simulink model "hopper_6dof_NED_v2_fswBridge"  (R2026a)
settings: Solver=FixedStepAuto  StopTime=30  FixedStep=1e-3  RelTol=1e-5
InitFcn:
  | if ~exist('SENS', 'var'), addpath(fullfile(fileparts(get_param(bdroot, 'FileName')), 'fsw_bridge')); SENS = sensor_params(); end
undefined symbols (not defined in the file): cg_init, dcg_dMfu_table, dcg_dMox_table, dI_dMfu_table, dI_dMox_table, ENGINE, engine_cg, engine_mass, fu_axial_damping_ratios, fu_lateral_damping_ratios, fu_mass_profile, fu_masses, fu_mdot_data, g, IN, K1flat, K2grid, MoI_init, mount_cg, OUT, ox_axial_damping_ratios, ox_lateral_damping_ratios, ox_mass_profile, ox_masses, ox_mdot_data, pressureLevels, r_leg_1, r_leg_2, r_leg_3, r_leg_4, tank_r, TANKS, Target_Trajectory, tgrid, thrust_data, unom, uwndTable, VEH, vwndTable
libraries: fl_lib x31, nesl_utility x25, matrix_library x18, SimscapeFluids_lib x10, simulink_extras x7, slpidlib x7, simulink x5, dspindex x3, sl_discontinuities x2, aerolibanim x1, commrandsrc3 x1, aerolibutil x1
(part 7 of 7)

== system hopper_6dof_NED_v2_fswBridge/Environment/Ground /Leg 1 Force2/If Action Subsystem ==
  Leg Position : Inport
  Leg Velocity : Inport  Port=2
  Action Port : ActionPort  ActionPortLabel=|
      | if(u1 > -0.001 
      | )
  Constant : Constant  Value=0.001
  Demux : Demux  Outputs=3
  Demux1 : Demux  Outputs=3
  Divide : Product  Inputs=*/
  Dot Product : DotProduct  OutDataTypeStr=Inherit: Inherit via internal rule
  Gain : Gain  Gain=-147150
  Gain1 : Gain  Gain=-7672.03
  Gain2 : Gain  Gain=-0.6
  Gain3 : Gain  Gain=-1
  Gain4 : Gain  Gain=-1
  Mux : Mux  Inputs=3
  Mux1 : Mux  Inputs=3
  Product : Product
  Sqrt : Sqrt
  Sum : Sum  Inputs=|++
  Sum1 : Sum  Inputs=|++
  Sum2 : Sum  Inputs=|++
  Zero : Constant  Value=0  OutDataTypeStr=Inherit: Inherit via back propagation
  Zero1 : Constant  Value=0  OutDataTypeStr=Inherit: Inherit via back propagation
  Zero2 : Constant  Value=0  OutDataTypeStr=Inherit: Inherit via back propagation
  Leg Force : Outport
  wires:
  Leg Position/1 -> Demux/1
  Leg Velocity/1 -> Demux1/1
  Gain/1 -> Sum/1
  Gain1/1 -> Sum/2
  Demux1/3 -> Gain1/1
  Demux1/2 -> Mux/2
  Demux1/1 -> Mux/1
  Mux/1 -> Dot Product/2, Dot Product/1, Divide/1
  Dot Product/1 -> Sqrt/1
  Divide/1 -> Product/2
  Gain2/1 -> Product/1
  Product/1 -> Gain4/1
  Sum1/1 -> Leg Force/1
  Sqrt/1 -> Sum2/1
  Sum2/1 -> Divide/2
  Constant/1 -> Sum2/2
  Sum/1 -> Gain3/1
  Zero1/1 -> Mux1/2
  Zero2/1 -> Mux1/3
  Mux1/1 -> Sum1/1, Gain2/1
  Demux/3 -> Gain/1
  Zero/1 -> Mux/3
  Gain3/1 -> Mux1/1
  Gain4/1 -> Sum1/2

== system hopper_6dof_NED_v2_fswBridge/Environment/Ground /Leg 1 Force2/If Action Subsystem1 ==
  Action Port : ActionPort  ActionPortLabel=else
  Constant : Constant  Value=[0 0 0]
  Out1 : Outport
  wires:
  Constant/1 -> Out1/1

== system hopper_6dof_NED_v2_fswBridge/Environment/Ground /Leg 1 Force3/If Action Subsystem ==
  Leg Position : Inport
  Leg Velocity : Inport  Port=2
  Action Port : ActionPort  ActionPortLabel=|
      | if(u1 > -0.001 
      | )
  Constant : Constant  Value=0.001
  Demux : Demux  Outputs=3
  Demux1 : Demux  Outputs=3
  Divide : Product  Inputs=*/
  Dot Product : DotProduct  OutDataTypeStr=Inherit: Inherit via internal rule
  Gain : Gain  Gain=-147150
  Gain1 : Gain  Gain=-7672.03
  Gain2 : Gain  Gain=-0.6
  Gain3 : Gain  Gain=-1
  Gain4 : Gain  Gain=-1
  Mux : Mux  Inputs=3
  Mux1 : Mux  Inputs=3
  Product : Product
  Sqrt : Sqrt
  Sum : Sum  Inputs=|++
  Sum1 : Sum  Inputs=|++
  Sum2 : Sum  Inputs=|++
  Zero : Constant  Value=0  OutDataTypeStr=Inherit: Inherit via back propagation
  Zero1 : Constant  Value=0  OutDataTypeStr=Inherit: Inherit via back propagation
  Zero2 : Constant  Value=0  OutDataTypeStr=Inherit: Inherit via back propagation
  Leg Force : Outport
  wires:
  Leg Position/1 -> Demux/1
  Leg Velocity/1 -> Demux1/1
  Gain/1 -> Sum/1
  Gain1/1 -> Sum/2
  Demux1/3 -> Gain1/1
  Demux1/2 -> Mux/2
  Demux1/1 -> Mux/1
  Mux/1 -> Dot Product/2, Dot Product/1, Divide/1
  Dot Product/1 -> Sqrt/1
  Divide/1 -> Product/2
  Gain2/1 -> Product/1
  Product/1 -> Gain4/1
  Sum1/1 -> Leg Force/1
  Sqrt/1 -> Sum2/1
  Sum2/1 -> Divide/2
  Constant/1 -> Sum2/2
  Sum/1 -> Gain3/1
  Zero1/1 -> Mux1/2
  Zero2/1 -> Mux1/3
  Mux1/1 -> Sum1/1, Gain2/1
  Demux/3 -> Gain/1
  Zero/1 -> Mux/3
  Gain3/1 -> Mux1/1
  Gain4/1 -> Sum1/2

== system hopper_6dof_NED_v2_fswBridge/Environment/Ground /Leg 1 Force3/If Action Subsystem1 ==
  Action Port : ActionPort  ActionPortLabel=else
  Constant : Constant  Value=[0 0 0]
  Out1 : Outport
  wires:
  Constant/1 -> Out1/1

== matlab function hopper_6dof_NED_v2_fswBridge/Environment/Slosh/Oxidizer Yaw Force/MATLAB Function ==
  data: ox_yaw_accel input; accel_term output; ox_lateral_pendulum_l input
function accel_term = fcn(ox_yaw_accel, ox_lateral_pendulum_l)

accel_term = -ox_yaw_accel / ox_lateral_pendulum_l;

end

== matlab function hopper_6dof_NED_v2_fswBridge/Environment/Slosh/Oxidizer Yaw Force/MATLAB Function1 ==
  data: ox_yaw_phi input; ang_term output; ox_lateral_natural_freq input
function ang_term = fcn(ox_yaw_phi, ox_lateral_natural_freq)

ang_term = -ox_lateral_natural_freq^2 * ox_yaw_phi;

end

== matlab function hopper_6dof_NED_v2_fswBridge/Environment/Slosh/Oxidizer Yaw Force/MATLAB Function2 ==
  data: ox_yaw_phi_dot input; velo_term output; ox_lateral_natural_freq input; ox_lateral_damping input
function velo_term = fcn(ox_yaw_phi_dot, ox_lateral_natural_freq,ox_lateral_damping)

velo_term = -2 * ox_lateral_damping * ox_lateral_natural_freq * ox_yaw_phi_dot;
end

== matlab function hopper_6dof_NED_v2_fswBridge/Environment/Slosh/Oxidizer Yaw Force/MATLAB Function3 ==
  data: ox_yaw_phi_ddot input; ox_yaw_f output; ox_lateral_slosh_mass input; ox_lateral_pendulum_l input
function ox_yaw_f = fcn(ox_yaw_phi_ddot, ox_lateral_slosh_mass, ox_lateral_pendulum_l)

ox_yaw_f = ox_lateral_slosh_mass * ox_lateral_pendulum_l * ox_yaw_phi_ddot;
end

== matlab function hopper_6dof_NED_v2_fswBridge/Environment/Slosh/Oxidizer Axial Force/MATLAB Function ==
  data: ox_axial_accel input; accel_term output; ox_axial_pendulum_l input
function accel_term = fcn(ox_axial_accel, ox_axial_pendulum_l)

accel_term = -ox_axial_accel / ox_axial_pendulum_l;

end

== matlab function hopper_6dof_NED_v2_fswBridge/Environment/Slosh/Oxidizer Axial Force/MATLAB Function1 ==
  data: ox_axial_phi input; ang_term output; ox_axial_natural_freq input
function ang_term = fcn(ox_axial_phi, ox_axial_natural_freq)

ang_term = -ox_axial_natural_freq^2 * ox_axial_phi;

end

== matlab function hopper_6dof_NED_v2_fswBridge/Environment/Slosh/Oxidizer Axial Force/MATLAB Function2 ==
  data: ox_axial_phi_dot input; velo_term output; ox_axial_natural_freq input; ox_axial_damping input
function velo_term = fcn(ox_axial_phi_dot, ox_axial_natural_freq,ox_axial_damping)

velo_term = -2 * ox_axial_damping * ox_axial_natural_freq * ox_axial_phi_dot;
end

== matlab function hopper_6dof_NED_v2_fswBridge/Environment/Slosh/Oxidizer Axial Force/MATLAB Function3 ==
  data: ox_axial_phi_ddot input; ox_axial_f output; ox_axial_slosh_mass input; ox_axial_pendulum_l input
function ox_axial_f = fcn(ox_axial_phi_ddot, ox_axial_slosh_mass, ox_axial_pendulum_l)

ox_axial_f = ox_axial_slosh_mass * ox_axial_pendulum_l * ox_axial_phi_ddot;
end

== matlab function hopper_6dof_NED_v2_fswBridge/Environment/Slosh/Fuel Axial Force/MATLAB Function ==
  data: fu_axial_accel input; accel_term output; fu_axial_pendulum_l input
function accel_term = fcn(fu_axial_accel, fu_axial_pendulum_l)

accel_term = -fu_axial_accel / fu_axial_pendulum_l;

end

== matlab function hopper_6dof_NED_v2_fswBridge/Environment/Slosh/Fuel Axial Force/MATLAB Function1 ==
  data: fu_axial_phi input; ang_term output; fu_axial_natural_freq input
function ang_term = fcn(fu_axial_phi, fu_axial_natural_freq)

ang_term = -fu_axial_natural_freq^2 * fu_axial_phi;

end

== matlab function hopper_6dof_NED_v2_fswBridge/Environment/Slosh/Fuel Axial Force/MATLAB Function2 ==
  data: fu_axial_phi_dot input; velo_term output; fu_axial_natural_freq input; fu_axial_damping input
function velo_term = fcn(fu_axial_phi_dot, fu_axial_natural_freq,fu_axial_damping)

velo_term = -2 * fu_axial_damping * fu_axial_natural_freq * fu_axial_phi_dot;
end

== matlab function hopper_6dof_NED_v2_fswBridge/Environment/Slosh/Fuel Axial Force/MATLAB Function3 ==
  data: fu_axial_phi_ddot input; fu_axial_f output; fu_axial_slosh_mass input; fu_axial_pendulum_l input
function fu_axial_f = fcn(fu_axial_phi_ddot, fu_axial_slosh_mass, fu_axial_pendulum_l)

fu_axial_f = fu_axial_slosh_mass * fu_axial_pendulum_l * fu_axial_phi_ddot;
end

== matlab function hopper_6dof_NED_v2_fswBridge/Environment/Slosh/Fuel Yaw Force/MATLAB Function ==
  data: fu_pitch_accel input; accel_term output; fu_lateral_pendulum_l input
function accel_term = fcn(fu_pitch_accel, fu_lateral_pendulum_l)

accel_term = -fu_pitch_accel / fu_lateral_pendulum_l;

end

== matlab function hopper_6dof_NED_v2_fswBridge/Environment/Slosh/Fuel Yaw Force/MATLAB Function1 ==
  data: fu_pitch_phi input; ang_term output; fu_lateral_natural_freq input
function ang_term = fcn(fu_pitch_phi, fu_lateral_natural_freq)

ang_term = -fu_lateral_natural_freq^2 * fu_pitch_phi;

end

== matlab function hopper_6dof_NED_v2_fswBridge/Environment/Slosh/Fuel Yaw Force/MATLAB Function2 ==
  data: fu_pitch_phi_dot input; velo_term output; fu_lateral_natural_freq input; fu_lateral_damping input
function velo_term = fcn(fu_pitch_phi_dot, fu_lateral_natural_freq,fu_lateral_damping)

velo_term = -2 * fu_lateral_damping * fu_lateral_natural_freq * fu_pitch_phi_dot;
end

== matlab function hopper_6dof_NED_v2_fswBridge/Environment/Slosh/Fuel Yaw Force/MATLAB Function3 ==
  data: fu_pitch_phi_ddot input; fu_pitch_f output; fu_lateral_slosh_mass input; fu_lateral_pendulum_l input
function fu_pitch_f = fcn(fu_pitch_phi_ddot, fu_lateral_slosh_mass, fu_lateral_pendulum_l)

fu_pitch_f = fu_lateral_slosh_mass * fu_lateral_pendulum_l * fu_pitch_phi_ddot;
end

== matlab function hopper_6dof_NED_v2_fswBridge/Environment/Slosh/Fuel Pitch Force/MATLAB Function ==
  data: fu_yaw_accel input; accel_term output; fu_lateral_pendulum_l input
function accel_term = fcn(fu_yaw_accel, fu_lateral_pendulum_l)

accel_term = -fu_yaw_accel / fu_lateral_pendulum_l;

end

== matlab function hopper_6dof_NED_v2_fswBridge/Environment/Slosh/MATLAB Function ==
  data: ox_lateral_natural_freq output; ox_axial_natural_freq output; ox_mass input; ox_lateral_slosh_mass output; ox_axial_slosh_mass output; ox_lateral_pendulum_l output; ox_aeff input; ox_axial_pendulum_l output; ox_lateral_damping output; ox_axial_damping output; tank_r input; ox_lateral_damping input; ox_axial_damping input
function [ox_lateral_natural_freq, ox_axial_natural_freq, ox_lateral_slosh_mass,ox_axial_slosh_mass, ox_lateral_pendulum_l, ox_axial_pendulum_l, ox_lateral_damping, ox_axial_damping]  = slosh_parameters(ox_mass, ox_aeff, tank_r, ox_lateral_damping, ox_axial_damping)

zeta = 1.841; % 1st eigen mode of oscillation for a cylindrical tank
ox_density = 1141;   % kg/m^3
% ox_tank_cg = 1.854; % m
% ox_tank_h =  TANKS.singular.oxidizer.h;
geff = norm(ox_aeff) + 0.001;

% Oxidizer Fluid
if ox_mass > 0.001
   h_ox_fluid = (ox_mass / ox_density) / (pi * tank_r^2);

   % Slosh Natural Frequencies
    ox_lateral_natural_freq = sqrt(zeta * geff / tank_r) * tanh(zeta * h_ox_fluid / tank_r);
    ox_axial_natural_freq = pi * sqrt(geff / h_ox_fluid);

    % Slosh Masses 
    ox_lateral_slosh_mass = ox_mass * (2 * tank_r * tanh(2 * zeta * h_ox_fluid / (2 * tank_r))) / (zeta * (zeta^2 - 1) * h_ox_fluid);
    ox_axial_slosh_mass = 1 / (pi^2) *  ox_mass;

    % Slosh Pendulum Lengths
    ox_lateral_pendulum_l = (2 * tank_r) / (2 * zeta * tanh(2*zeta * h_ox_fluid / (2 * tank_r)));
    ox_axial_pendulum_l = geff / ox_axial_natural_freq^2;
else
   h_ox_fluid = 0; 
   ox_lateral_natural_freq = 0;
   ox_axial_natural_freq = 0;
   ox_lateral_slosh_mass = 0;
   ox_axial_slosh_mass = 0;
   ox_lateral_pendulum_l = 1;
   ox_axial_pendulum_l = 1;
end



end

== matlab function hopper_6dof_NED_v2_fswBridge/Environment/Slosh/Fuel Pitch Force/MATLAB Function1 ==
  data: fu_yaw_phi input; ang_term output; fu_lateral_natural_freq input
function ang_term = fcn(fu_yaw_phi, fu_lateral_natural_freq)

ang_term = -fu_lateral_natural_freq^2 * fu_yaw_phi;

end

== matlab function hopper_6dof_NED_v2_fswBridge/Environment/Slosh/Fuel Pitch Force/MATLAB Function2 ==
  data: fu_yaw_phi_dot input; velo_term output; fu_lateral_natural_freq input; fu_lateral_damping input
function velo_term = fcn(fu_yaw_phi_dot, fu_lateral_natural_freq, fu_lateral_damping)

velo_term = -2 * fu_lateral_damping * fu_lateral_natural_freq * fu_yaw_phi_dot;
end

== matlab function hopper_6dof_NED_v2_fswBridge/Environment/Slosh/Fuel Pitch Force/MATLAB Function3 ==
  data: fu_yaw_phi_ddot input; fu_yaw_f output; fu_lateral_slosh_mass input; fu_lateral_pendulum_l input
function fu_yaw_f = fcn(fu_yaw_phi_ddot, fu_lateral_slosh_mass, fu_lateral_pendulum_l)

fu_yaw_f = fu_lateral_slosh_mass * fu_lateral_pendulum_l * fu_yaw_phi_ddot;
end

== matlab function hopper_6dof_NED_v2_fswBridge/Environment/CG // MOI Script v3/MATLAB Function ==
  data: r_ox input; I_m_ox output
function I_m_ox = fcn(r_ox)
x = r_ox(1);
y = r_ox(2);
z = r_ox(3);

I_m_ox = [y^2 + z^2 -x*y x*z;
       -x*y x^2 + z^2 -y*z;
       -x*z y*z  x^2 + y^2
    ];

== matlab function hopper_6dof_NED_v2_fswBridge/Environment/CG // MOI Script v3/MATLAB Function1 ==
  data: r_fu input; I_m_fu output
function I_m_fu = fcn(r_fu)
x = r_fu(1);
y = r_fu(2);
z = r_fu(3);

I_m_fu = [y^2 + z^2 -x*y x*z;
       -x*y x^2 + z^2 -y*z;
       -x*z y*z  x^2 + y^2
    ];

== matlab function hopper_6dof_NED_v2_fswBridge/Environment/Slosh/Oxidizer Axial Force/MATLAB Function4 ==
  data: x_omega_dot input; x_slosh_torque output; ox_axial_slosh_mass input; ox_axial_pendulum_l input; slosh_angular_accel input
function x_slosh_torque = fcn(x_omega_dot, ox_axial_slosh_mass, ox_axial_pendulum_l, slosh_angular_accel)

I_s = ox_axial_slosh_mass * ox_axial_pendulum_l^2;

x_slosh_torque = -I_s*(x_omega_dot - slosh_angular_accel);

== matlab function hopper_6dof_NED_v2_fswBridge/Environment/Slosh/Fuel Axial Force/MATLAB Function4 ==
  data: x_omega_dot input; x_slosh_torque output; fu_axial_slosh_mass input; fu_axial_pendulum_l input; slosh_angular_accel input
function x_slosh_torque = fcn(x_omega_dot, fu_axial_slosh_mass, fu_axial_pendulum_l, slosh_angular_accel)

I_s = fu_axial_slosh_mass * fu_axial_pendulum_l^2;

x_slosh_torque = -I_s*(x_omega_dot - slosh_angular_accel);

== matlab function hopper_6dof_NED_v2_fswBridge/Environment/Slosh/Oxidizer Yaw Force/MATLAB Function4 ==
  data: y_omega_dot input; y_slosh_torque output; ox_lateral_slosh_mass input; ox_lateral_pendulum_l input; slosh_angular_accel input
function y_slosh_torque = fcn(y_omega_dot, ox_lateral_slosh_mass, ox_lateral_pendulum_l, slosh_angular_accel)

I_s = ox_lateral_slosh_mass * ox_lateral_pendulum_l^2;

y_slosh_torque = -I_s*(y_omega_dot - slosh_angular_accel);

== matlab function hopper_6dof_NED_v2_fswBridge/Environment/Slosh/Fuel Yaw Force/MATLAB Function4 ==
  data: y_omega_dot input; y_slosh_torque output; fu_lateral_slosh_mass input; fu_lateral_pendulum_l input; slosh_angular_accel input
function y_slosh_torque = fcn(y_omega_dot, fu_lateral_slosh_mass, fu_lateral_pendulum_l, slosh_angular_accel)

I_s = fu_lateral_slosh_mass * fu_lateral_pendulum_l^2;

y_slosh_torque = -I_s*(y_omega_dot - slosh_angular_accel);

== matlab function hopper_6dof_NED_v2_fswBridge/Environment/Slosh/Oxidizer Pitch Force/MATLAB Function4 ==
  data: z_omega_dot input; z_slosh_torque output; ox_lateral_slosh_mass input; ox_lateral_pendulum_l input; slosh_angular_accel input
function z_slosh_torque = fcn(z_omega_dot, ox_lateral_slosh_mass, ox_lateral_pendulum_l, slosh_angular_accel)

I_s = ox_lateral_slosh_mass * ox_lateral_pendulum_l^2;

z_slosh_torque = -I_s*(z_omega_dot - slosh_angular_accel);

== matlab function hopper_6dof_NED_v2_fswBridge/Environment/Slosh/Fuel Pitch Force/MATLAB Function4 ==
  data: z_omega_dot input; z_slosh_torque output; fu_lateral_slosh_mass input; fu_lateral_pendulum_l input; slosh_angular_accel input
function z_slosh_torque = fcn(z_omega_dot, fu_lateral_slosh_mass, fu_lateral_pendulum_l, slosh_angular_accel)

I_s = fu_lateral_slosh_mass * fu_lateral_pendulum_l^2;

z_slosh_torque = -I_s*(z_omega_dot - slosh_angular_accel);

== matlab function hopper_6dof_NED_v2_fswBridge/Environment/CG // MOI Script v3/MATLAB Function2 ==
  data: delta_y input; rot_mat output; delta_z input
function rot_mat = fcn(delta_y, delta_z)

rot_mat = [0 -delta_z delta_y;
           delta_z 0 0;
           -delta_y 0 0];

== matlab function hopper_6dof_NED_v2_fswBridge/Environment/Sensors/imu_model ==
  settings: updateMethod=DISCRETE  sampleTime=SENS.imu.Ts
  data: F_b input; imu output; W_b input; mass input; w_b input; SENS parameter
function imu = imu_model(F_b, W_b, mass, w_b, SENS)
%#codegen
% IMU measurement model (Notion: IMU Measurement Model), ADIS16500.
%   F_b  total force on the vehicle, body axes (N)
%   W_b  weight, body axes (N)
%   mass vehicle mass (kg)
%   w_b  body angular rate (rad/s)
%   imu  [accel (3) m/s^2; gyro (3) deg/s], sensor axes
%
%   f = (I+Ma)(I+Sa) Rbs f_true + ba + na
%   w = (I+Mg)(I+Sg) Rbs w_true + Gg Rbs f_true + bg + ng
%   Biases = turn-on offset (drawn once) + first-order Gauss-Markov drift.
P = SENS.imu;
persistent s ba0 bg0 bad bgd Sa Sg Ma Mg
if isempty(s)
    s = rng_seed(SENS.seed, 1);
    [n, s] = rng_gauss(s, 3); ba0 = P.acc_b0_sd * n;
    [n, s] = rng_gauss(s, 3); bg0 = P.gyro_b0_sd * n;
    [n, s] = rng_gauss(s, 3); bad = P.acc_b_sd * n;
    [n, s] = rng_gauss(s, 3); bgd = P.gyro_b_sd * n;
    [n, s] = rng_gauss(s, 3); Sa = diag(1 + P.sf_sd * n);
    [n, s] = rng_gauss(s, 3); Sg = diag(1 + P.sf_sd * n);
    [n, s] = rng_gauss(s, 6); Ma = eye(3) + P.misalign_sd * [0 n(1) n(2); n(3) 0 n(4); n(5) n(6) 0];
    [n, s] = rng_gauss(s, 6); Mg = eye(3) + P.misalign_sd * [0 n(1) n(2); n(3) 0 n(4); n(5) n(6) 0];
end

% Specific force at the CG, plus centripetal term at the sensor location
f_true = (F_b(:) - W_b(:)) / mass + cross(w_b(:), cross(w_b(:), P.r_b));
f_s = P.R_bs * f_true;
w_s = P.R_bs * w_b(:);

% Gauss-Markov bias drift
phi_a = exp(-P.Ts / P.acc_b_tau);
phi_g = exp(-P.Ts / P.gyro_b_tau);
[n, s] = rng_gauss(s, 3); bad = phi_a * bad + sqrt(1 - phi_a^2) * P.acc_b_sd * n;
[n, s] = rng_gauss(s, 3); bgd = phi_g * bgd + sqrt(1 - phi_g^2) * P.gyro_b_sd * n;

% White noise, per-sample sd from the noise density
[na, s] = rng_gauss(s, 3);
[ng, s] = rng_gauss(s, 3);
f_meas = Ma * Sa * f_s + ba0 + bad + P.acc_nd / sqrt(P.Ts) * na;
w_meas = Mg * Sg * w_s + P.g_sens * f_s + bg0 + bgd + P.gyro_nd / sqrt(P.Ts) * ng;

imu = [f_meas; w_meas * (180 / pi)];
end

% --- deterministic RNG shared by the sensor blocks (xorshift32 + Box-Muller)
% Same numbers in Simulink and in generated C, seeded per run and per sensor.
function s = rng_seed(seed, stream)
s = uint32(mod(double(seed) * 2654435761 + double(stream) * 97531 + 12345, 4294967296));
if s == 0
    s = uint32(1);
end
end

function [u, s] = rng_uniform(s)
s = bitxor(s, bitshift(s, 13));
s = bitxor(s, bitshift(s, -17));
s = bitxor(s, bitshift(s, 5));
u = (double(s) + 0.5) / 4294967296;
end

function [n, s] = rng_gauss(s, k)
n = zeros(k, 1);
for i = 1:k
    [u1, s] = rng_uniform(s);
    [u2, s] = rng_uniform(s);
    n(i) = sqrt(-2 * log(u1)) * cos(2 * pi * u2);
end
end

== matlab function hopper_6dof_NED_v2_fswBridge/Environment/Sensors/mag_model ==
  settings: updateMethod=DISCRETE  sampleTime=SENS.mag.Ts
  data: C_bn input; mag output; SENS parameter
function mag = mag_model(C_bn, SENS)
%#codegen
% Magnetometer measurement model (Notion: Magnetometer Model), LIS2MDL.
%   C_bn NED -> body rotation (6DOF DCMbe)
%   mag  magnetic field, sensor axes, Gauss
%
%   z = A Cbn Bn + beta + eta
%   A folds soft iron, scale factor and misalignment; beta is hard iron.
%   Both are drawn once per run (they are what calibration estimates).
P = SENS.mag;
persistent s A beta
if isempty(s)
    s = rng_seed(SENS.seed, 2);
    [n, s] = rng_gauss(s, 9); A = eye(3) + P.A_sd * reshape(n, 3, 3);
    [n, s] = rng_gauss(s, 3); beta = P.beta_sd * n;
end

[n, s] = rng_gauss(s, 3);
mag = A * (C_bn * P.B_n) + beta + P.noise_sd * n;
end

% --- deterministic RNG shared by the sensor blocks (xorshift32 + Box-Muller)
function s = rng_seed(seed, stream)
s = uint32(mod(double(seed) * 2654435761 + double(stream) * 97531 + 12345, 4294967296));
if s == 0
    s = uint32(1);
end
end

function [u, s] = rng_uniform(s)
s = bitxor(s, bitshift(s, 13));
s = bitxor(s, bitshift(s, -17));
s = bitxor(s, bitshift(s, 5));
u = (double(s) + 0.5) / 4294967296;
end

function [n, s] = rng_gauss(s, k)
n = zeros(k, 1);
for i = 1:k
    [u1, s] = rng_uniform(s);
    [u2, s] = rng_uniform(s);
    n(i) = sqrt(-2 * log(u1)) * cos(2 * pi * u2);
end
end

== matlab function hopper_6dof_NED_v2_fswBridge/Environment/Sensors/baro_model ==
  settings: updateMethod=DISCRETE  sampleTime=SENS.baro.Ts
  data: p_n input; baro output; v_n input; C_bn input; thrust input; SENS parameter
function baro = baro_model(p_n, v_n, C_bn, thrust, SENS)
%#codegen
% Barometer measurement model (Notion: Barometer Model), MS5611.
%   p_n    CG position NED (m), ground at D = 0
%   v_n    CG velocity NED (m/s)
%   C_bn   NED -> body rotation
%   thrust delivered thrust (N); > 0 means the engine is on
%   baro   [pressure Pa; temperature degC]
%
%   p = p_atm(h) + dp_ground_effect(h) + dp_dynamic + beta + eta, quantized
%   Tare/zeroing is left to the flight software.
P = SENS.baro;
persistent s b
if isempty(s)
    s = rng_seed(SENS.seed, 3);
    [n, s] = rng_gauss(s, 1); b = P.b0_sd * n;
end

% Height of the sensor port above the pad
r_n = C_bn' * P.r_b;
h = -(p_n(3) + r_n(3));

% Standard atmosphere from the pad conditions
T = P.T_pad - P.L * h;
p_atm = P.p_pad * (T / P.T_pad)^(P.g0 / (P.L * P.R));

% Exhaust ground effect, only near the pad with the engine on
dp_ge = 0;
if thrust > 0 && h < P.ge_D
    dp_ge = P.ge_sign * P.ge_A * (P.ge_D - max(h, 0))^2;
end

% Part of the dynamic pressure reaching the port
rho = p_atm / (P.R * T);
v_rel = v_n(:) - P.wind_n;
dp_dyn = P.k_port * 0.5 * rho * (v_rel' * v_rel);

% Gauss-Markov bias drift and white noise
phi = exp(-P.Ts / P.b_tau);
[n, s] = rng_gauss(s, 2);
b = phi * b + sqrt(1 - phi^2) * P.b_sd * n(1);
p = p_atm + dp_ge + dp_dyn + b + P.noise_sd * n(2);

baro = [P.dq * round(p / P.dq); T - 273.15];
end

% --- deterministic RNG shared by the sensor blocks (xorshift32 + Box-Muller)
function s = rng_seed(seed, stream)
s = uint32(mod(double(seed) * 2654435761 + double(stream) * 97531 + 12345, 4294967296));
if s == 0
    s = uint32(1);
end
end

function [u, s] = rng_uniform(s)
s = bitxor(s, bitshift(s, 13));
s = bitxor(s, bitshift(s, -17));
s = bitxor(s, bitshift(s, 5));
u = (double(s) + 0.5) / 4294967296;
end

function [n, s] = rng_gauss(s, k)
n = zeros(k, 1);
for i = 1:k
    [u1, s] = rng_uniform(s);
    [u2, s] = rng_uniform(s);
    n(i) = sqrt(-2 * log(u1)) * cos(2 * pi * u2);
end
end

== matlab function hopper_6dof_NED_v2_fswBridge/Environment/Sensors/gps_model ==
  settings: updateMethod=DISCRETE  sampleTime=SENS.gps.tick
  data: p_n input; gps output; v_n input; C_bn input; w_b input; thrust input; SENS parameter
function gps = gps_model(p_n, v_n, C_bn, w_b, thrust, SENS)
%#codegen
% GPS measurement model (Notion: GPS Measurement Model), u-blox ZED-F9P.
%   p_n, v_n  CG position (m) and velocity (m/s), NED from the pad
%   C_bn      NED -> body rotation
%   w_b       body angular rate (rad/s)
%   thrust    delivered thrust (N); engine on raises the dropout chance
%   gps       [lat deg; lon deg; alt m; vN; vE; vD m/s; has_fix; num_sats]
%             (luna GpsState fields)
%
%   p = p_cg + Cbn' r_b + b_slow + b_fast + eta_p
%   v = v_cg + Cbn' (w x r_b) + eta_v
%   Drifts are unit Gauss-Markov states scaled by the mode's sigmas. Each fix
%   is converted to lat/lon/height, quantized, and delivered `latency` later.
%   Runs every `tick` seconds so fix times and latency land on the grid.
%   Not modelled yet: pad multipath, RTK fixed/float transitions.
P = SENS.gps;
m = P.mode + 1;
persistent s zs zf out pend pend_at k fix
if isempty(s)
    s = rng_seed(SENS.seed, 4);
    [zs, s] = rng_gauss(s, 3);
    [zf, s] = rng_gauss(s, 3);
    out = zeros(8, 1);          % nothing received yet: has_fix = 0
    pend = zeros(8, 1);
    pend_at = -1;
    k = 0;
    fix = true;
end

Tg = 1 / P.rate;
n_fix = round(Tg / P.tick);
n_lat = round(P.latency / P.tick);

if mod(k, n_fix) == 0
    % Drift states advance once per fix
    phs = exp(-Tg / P.tau_slow(m));
    phf = exp(-Tg / P.tau_fast(m));
    [n, s] = rng_gauss(s, 3); zs = phs * zs + sqrt(1 - phs^2) * n;
    [n, s] = rng_gauss(s, 3); zf = phf * zf + sqrt(1 - phf^2) * n;

    % Fix lost / regained
    [u, s] = rng_uniform(s);
    if fix
        p_loss = P.p_loss(1);
        if thrust > 0
            p_loss = P.p_loss(2);
        end
        fix = u >= p_loss;
    else
        fix = u < 1 - exp(-Tg / P.T_reacq);
    end

    [np, s] = rng_gauss(s, 3);
    [nv, s] = rng_gauss(s, 3);
    if fix
        dH = P.dop_scale(1);
        dV = P.dop_scale(2);
        C_nb = C_bn';
        pos = p_n(:) + C_nb * P.r_b ...
            + [P.sH_slow(m) * dH; P.sH_slow(m) * dH; P.sV_slow(m) * dV] .* zs ...
            + [P.sH_fast(m) * dH; P.sH_fast(m) * dH; P.sV_fast(m) * dV] .* zf ...
            + [P.sH_white(m) * dH; P.sH_white(m) * dH; P.sV_white(m) * dV] .* np;
        vel = v_n(:) + C_nb * cross(w_b(:), P.r_b) + [P.svH * dH; P.svH * dH; P.svD * dV] .* nv;

        % NED metres from the pad -> geodetic (flat Earth over the flight)
        a = 6378137;
        e2 = 0.00669438;
        lat0 = P.lat0 * pi / 180;
        sl2 = sin(lat0)^2;
        N0 = a / sqrt(1 - e2 * sl2);
        RM = a * (1 - e2) / (1 - e2 * sl2)^1.5;
        lat = P.lat0 + pos(1) / (RM + P.h0) * 180 / pi;
        lon = P.lon0 + pos(2) / ((N0 + P.h0) * cos(lat0)) * 180 / pi;
        alt = P.h0 - pos(3);

        q = P.dq_deg(m);
        qa = P.dq_alt(m);
        pend = [q * round(lat / q); q * round(lon / q); qa * round(alt / qa); ...
                P.dq_vel * round(vel / P.dq_vel); 1; P.num_sats];
    else
        pend = [out(1:6); 0; 0];  % no new solution; last values held
    end
    pend_at = k + n_lat;
end

if k == pend_at
    out = pend;
end
k = k + 1;
gps = out;
end

% --- deterministic RNG shared by the sensor blocks (xorshift32 + Box-Muller)
function s = rng_seed(seed, stream)
s = uint32(mod(double(seed) * 2654435761 + double(stream) * 97531 + 12345, 4294967296));
if s == 0
    s = uint32(1);
end
end

function [u, s] = rng_uniform(s)
s = bitxor(s, bitshift(s, 13));
s = bitxor(s, bitshift(s, -17));
s = bitxor(s, bitshift(s, 5));
u = (double(s) + 0.5) / 4294967296;
end

function [n, s] = rng_gauss(s, k)
n = zeros(k, 1);
for i = 1:k
    [u1, s] = rng_uniform(s);
    [u2, s] = rng_uniform(s);
    n(i) = sqrt(-2 * log(u1)) * cos(2 * pi * u2);
end
end

== matlab function hopper_6dof_NED_v2_fswBridge/Environment/Sensors/lidar_model ==
  settings: updateMethod=DISCRETE  sampleTime=SENS.lidar.Ts
  data: p_n input; lidar output; C_bn input; SENS parameter
function lidar = lidar_model(p_n, C_bn, SENS)
%#codegen
% LiDAR measurement model, 4x Benewake TF-Luna (simplified).
%   p_n    CG position NED (m), ground plane at D = 0
%   C_bn   NED -> body rotation
%   lidar  range along each beam (m), -1 when there is no valid return
%
%   Range from each sensor along its beam to the flat ground, with
%   range-dependent noise, 1 cm steps, the datasheet range window and random
%   dropouts. Stand-in until the ray-traced model on Notion (plume, dust,
%   surface reflectivity) is implemented.
P = SENS.lidar;
persistent s
if isempty(s)
    s = rng_seed(SENS.seed, 5);
end

C_nb = C_bn';
lidar = -ones(4, 1);
for i = 1:4
    pos = p_n(:) + C_nb * P.r_b(:, i);
    d = C_nb * P.d_b(:, i);
    h = -pos(3);
    [u, s] = rng_uniform(s);
    [n, s] = rng_gauss(s, 1);
    if d(3) > 1e-6 && h > 0
        R = h / d(3);
        if R >= P.r_min && R <= P.r_max && u >= P.p_drop
            sd = P.sd_near;
            if R > 3
                sd = P.sd_frac * R;
            end
            lidar(i) = P.dq * round((R + sd * n) / P.dq);
        end
    end
end
end

% --- deterministic RNG shared by the sensor blocks (xorshift32 + Box-Muller)
function s = rng_seed(seed, stream)
s = uint32(mod(double(seed) * 2654435761 + double(stream) * 97531 + 12345, 4294967296));
if s == 0
    s = uint32(1);
end
end

function [u, s] = rng_uniform(s)
s = bitxor(s, bitshift(s, 13));
s = bitxor(s, bitshift(s, -17));
s = bitxor(s, bitshift(s, 5));
u = (double(s) + 0.5) / 4294967296;
end

function [n, s] = rng_gauss(s, k)
n = zeros(k, 1);
for i = 1:k
    [u1, s] = rng_uniform(s);
    [u2, s] = rng_uniform(s);
    n(i) = sqrt(-2 * log(u1)) * cos(2 * pi * u2);
end
end

== matlab function hopper_6dof_NED_v2_fswBridge/Environment/Fluid Network2/Fuel Throttle Valve Controller/Feed Forward ==
  data: mdot input; theta output; ptank input; pset input; rho input; CdA output
function [theta, CdA] = feed_forward(mdot,ptank,pset,rho)

dp = max(ptank - pset, 1e-6); % divide by zero error
CdA = mdot / sqrt(2*dp*rho);

CdA = max(CdA, 1e-7); % divide by zero error
Cv_vector = [1e-8, 0.01, 0.06, 0.21, 0.46, 0.83, 1.35, 2.04, 2.93];
CdA_vector = Cv_vector ./ 37.97;
theta_vector = 0.9.*[20,30,40,50,60,70,80,90,100];

theta = interp1(CdA_vector, theta_vector, CdA);
theta = min(theta, 90);
theta = max(theta, 0);
end

== matlab function hopper_6dof_NED_v2_fswBridge/Environment/Fluid Network2/Fuel Throttle Valve Controller/MATLAB Function5 ==
  data: time input; rate_limit_up output; rate_limit_down output
function [rate_limit_up, rate_limit_down] = fcn(time)
if time < 0.5
    rate_limit_up = 1350;
else
    rate_limit_up = 40;
end
rate_limit_down = -rate_limit_up;

== matlab function hopper_6dof_NED_v2_fswBridge/Controller ==
  data: t input; u output; x input; tgrid input; xref input; K1flat input; K2grid input; unom input
function u = Gain_Selector(t, x, tgrid, xref, K1flat, K2grid, unom)
%#codegen
% Fixed-size output: u is always 4x1

u = zeros(4,1);

x = x(:);              % should be 13x1 for 6DOF
N = length(tgrid);

% --- Clamp time and compute interval index ---
if t <= tgrid(1)
    idx = 1;
    w = 0.0;
elseif t >= tgrid(end)
    idx = N-1;
    w = 1.0;
else
    idx = 1;
    for k = 1:(N-1)
        if tgrid(k) <= t && t < tgrid(k+1)
            idx = k;
            break;
        end
    end
    t1 = tgrid(idx);
    t2 = tgrid(idx+1);
    w  = (t - t1) / (t2 - t1);
end

% --- Interpolate reference state (13x1) ---
xref_t = (1-w)*xref(idx,:)' + w*xref(idx+1,:)';

% --- Interpolate K1flat then reshape to 4x13 ---
Kflat = (1-w)*K1flat(idx,:) + w*K1flat(idx+1,:);
K1 = reshape(Kflat, 13, 4)';   % 4x13   (requires K1flat is N×52)

% --- Interpolate K2 (4x1) ---
K2 = (1-w)*K2grid(idx,:)' + w*K2grid(idx+1,:)';

% --- Interpolate nominal control (4x1) ---
u_nom = (1-w)*unom(idx,:)' + w*unom(idx+1,:)';

q     = x(10:13);
qref  = xref_t(10:13);

if dot(q,qref) < 0
    q = -q;
end

x_used = x;
x_used(10:13) = q;

dx = x_used - xref_t;


% --- Control law ---
%dx = (x - xref_t);          % 13x1
u  =u_nom+(-K1*dx)-K2;  
%fix

end

== matlab function hopper_6dof_NED_v2_fswBridge/Environment/Fluid Network2/Fuel Throttle Valve Controller/System ==
  data: Ptank input; CdA input; mdot input; Pout output; rho input; dp output
function [Pout,dp] = theta_to_pressure(Ptank,CdA,mdot, rho)

% CdA = mdot/(sqrt((2*(ptank-pout)*rho)

%CdA = max(CdA, 1e-7);
dp = (mdot/CdA)^2*1/(2*rho);

% (mdot/CdA)^2*rho/2 is solving for the pout from the dp in CdA eqn
Pout = Ptank - dp;
Pout = max(Pout, 0);

== matlab function hopper_6dof_NED_v2_fswBridge/Environment/Fluid Network2/MATLAB Function ==
  data: mdot_ox input; mdot_fuel input; eta_cstar input; Cf input; thrust output; Pc output; MR output; cstar_ideal input
function [thrust, Pc, MR] = engine_model(mdot_ox, mdot_fuel, eta_cstar, Cf, cstar_ideal)
%#codegen
% ENGINE_MODEL
%
% Inputs:
%   mdot_ox      - oxidizer mass flow rate [kg/s]
%   mdot_fuel    - fuel mass flow rate [kg/s]
%   eta_cstar    - c* efficiency [-]
%   Cf           - thrust coefficient [-]
%
% Outputs:
%   thrust       - thrust [N]
%   Pc           - chamber pressure [Pa]
%   MR           - mixture ratio [-]

    %% -------------------------
    % CONSTANTS
    % -------------------------
    At = 0.0008271;      % throat area [m^2]

    %% -------------------------
    % 1. Total mass flow
    % -------------------------
    mdot = mdot_ox + mdot_fuel;

    %% -------------------------
    % 2. Mixture ratio
    % -------------------------
    if mdot_fuel > 0
        MR = mdot_ox / mdot_fuel;
    else
        MR = 0; % avoid divide by zero
    end

    %% -------------------------
    % 3. Actual c*
    % -------------------------
    cstar_actual = eta_cstar * cstar_ideal;

    %% -------------------------
    % 4. Chamber pressure
    % -------------------------
    Pc = (mdot * cstar_actual) / At;

    %% -------------------------
    % 6. Thrust
    % -------------------------
    thrust = Cf * Pc * At;

    % Equivalent:
    % thrust = Cf * mdot * cstar_actual;

end

== matlab function hopper_6dof_NED_v2_fswBridge/Environment/Fluid Network2/Ox Throttle Valve Controller/Feed Forward ==
  data: mdot input; theta output; ptank input; pset input; rho input; CdA output
function [theta, CdA] = feed_forward(mdot,ptank,pset,rho)

dp = max(ptank - pset, 1e-6); % divide by zero error
CdA = mdot / sqrt(2*dp*rho);

CdA = max(CdA, 1e-7); % divide by zero error
Cv_vector = [1e-8, 0.01, 0.06, 0.21, 0.46, 0.83, 1.35, 2.04, 2.93];
CdA_vector = Cv_vector ./ 37.97;
theta_vector = 0.9.*[20,30,40,50,60,70,80,90,100];

theta = interp1(CdA_vector, theta_vector, CdA);
theta = min(theta, 90);
theta = max(theta, 0);
end

== matlab function hopper_6dof_NED_v2_fswBridge/Environment/Fluid Network2/Ox Throttle Valve Controller/MATLAB Function5 ==
  data: time input; rate_limit_up output; rate_limit_down output
function [rate_limit_up, rate_limit_down] = fcn(time)
if time < 0.5
    rate_limit_up = 1350;
else
    rate_limit_up = 40;
end
rate_limit_down = -rate_limit_up;

== matlab function hopper_6dof_NED_v2_fswBridge/Environment/Fluid Network2/Ox Throttle Valve Controller/System ==
  data: Ptank input; CdA input; mdot input; Pout output; rho input; dp output
function [Pout,dp] = theta_to_pressure(Ptank,CdA,mdot, rho)

% CdA = mdot/(sqrt((2*(ptank-pout)*rho)

%CdA = max(CdA, 1e-7);
dp = (mdot/CdA)^2*1/(2*rho);

% (mdot/CdA)^2*rho/2 is solving for the pout from the dp in CdA eqn
Pout = Ptank - dp;
Pout = max(Pout, 0);

== matlab function hopper_6dof_NED_v2_fswBridge/Environment/Fluid Network2/Thrust Commanded to mdot + bunch of other bs ==
  data: mdot_fuel output; rho_fuel_eng output; pc output; F_cmd input; rho_ox input; rho_fuel input; rho_ox_eng output; mdot_ox output; Cf input; MR input; cstar_ideal input; cstar_eff input
function [mdot_fuel, rho_fuel_eng, pc, rho_ox_eng, mdot_ox] = thrust_to_mdot( ...
   F_cmd, rho_ox, rho_fuel, Cf, MR, cstar_ideal, cstar_eff)
%#codegen
% Convert commanded thrust into mdots and convert densities to English units
%
% Outputs:
%   mdot_ox        - oxidizer mass flow rate [kg/s]
%   mdot_fuel      - fuel mass flow rate [kg/s]
%   rho_ox_eng     - oxidizer density [lb/ft^3]
%   rho_fuel_eng   - fuel density [lb/ft^3]
%   mdot_ox_lb     - oxidizer mass flow rate [lb/s]
%   mdot_fuel_lb   - fuel mass flow rate [lb/s]

    cstar = cstar_ideal * cstar_eff;
    At = 0.0008271;      % throat area [m^2]

    %% ---- DEFAULT OUTPUTS ----
    mdot_ox = 0;
    mdot_fuel = 0;
    rho_ox_eng = 0;
    rho_fuel_eng = 0;
    mdot_ox_lb = 0;
    mdot_fuel_lb = 0;

    %% ---- UNIT CONVERSION ----
    kgm3_to_lbft3 = 0.062428;
    kg_to_lb = 2.20462;

    rho_ox_eng = rho_ox * kgm3_to_lbft3;
    rho_fuel_eng = rho_fuel * kgm3_to_lbft3;

    %% ---- EFFECTIVE EXHAUST VELOCITY ----
    ve = Cf * cstar;


    %% ---- TOTAL MASS FLOW ----
    mdot_total = F_cmd / ve;

    pc = mdot_total * cstar / At;

    pc = pc * 0.000145038;

    %% ---- SPLIT BY MR ----
    mdot_ox = mdot_total * MR / (1 + MR);
    mdot_fuel = mdot_total / (1 + MR);


end

== matlab function hopper_6dof_NED_v2_fswBridge/Environment/Slosh/MATLAB Function1 ==
  data: fu_mass input; fu_lateral_natural_freq output; fu_axial_natural_freq output; fu_lateral_slosh_mass output; fu_aeff input; fu_axial_slosh_mass output; fu_lateral_pendulum_l output; fu_axial_pendulum_l output; fu_lateral_damping output; fu_axial_damping output; tank_r input; fu_lateral_damping input; fu_axial_damping input
function [fu_lateral_natural_freq, fu_axial_natural_freq, fu_lateral_slosh_mass, fu_axial_slosh_mass, fu_lateral_pendulum_l, fu_axial_pendulum_l, fu_lateral_damping, fu_axial_damping]  = slosh_parameters(fu_mass, fu_aeff, tank_r, fu_lateral_damping, fu_axial_damping) 
zeta = 1.841; % 1st eigen mode of oscillation for a cylindrical tank
fu_density = 800;    % kg/m^3
% fu_tank_cg = 1.0668; % m
% fu_tank_h = TANKS.singular.fuel.h;
geff = norm(fu_aeff) + 0.001;

if fu_mass > 0.001
   h_fu_fluid = (fu_mass / fu_density) / (pi * tank_r^2);
   % Fluid sits at the bottom of the tank shell
   % z_fu_fluid = (fu_tank_cg - fu_tank_h/2) + (h_fu_fluid / 2);

   % Slosh Natural Frequencies
    fu_lateral_natural_freq = sqrt(zeta * geff / tank_r) * tanh(zeta * h_fu_fluid / tank_r);
    fu_axial_natural_freq = pi * sqrt(geff / h_fu_fluid);

    % Slosh Masses 
    fu_lateral_slosh_mass = fu_mass * (2 * tank_r * tanh(2 * zeta * h_fu_fluid / (2 * tank_r))) / (zeta * (zeta^2 - 1) * h_fu_fluid);
    fu_axial_slosh_mass = 1 / (pi^2) *  fu_mass;

    % Slosh Pendulum Lengths
    fu_lateral_pendulum_l = (2 * tank_r) / (2 * zeta * tanh(2*zeta * h_fu_fluid / (2 * tank_r)));
    fu_axial_pendulum_l = geff / fu_axial_natural_freq^2;
else
   h_fu_fluid = 0;
   fu_lateral_natural_freq = 0;
   fu_axial_natural_freq = 0;
   fu_lateral_slosh_mass = 0;
   fu_axial_slosh_mass = 0;
   fu_lateral_pendulum_l = 1;
   fu_axial_pendulum_l = 1;
end





end

== matlab function hopper_6dof_NED_v2_fswBridge/Environment/Slosh/Oxidizer Pitch Force/MATLAB Function ==
  data: ox_pitch_accel input; accel_term output; ox_lateral_pendulum_l input
function accel_term = fcn(ox_pitch_accel, ox_lateral_pendulum_l)

accel_term = -ox_pitch_accel / ox_lateral_pendulum_l;

end

== matlab function hopper_6dof_NED_v2_fswBridge/Environment/Slosh/Oxidizer Pitch Force/MATLAB Function1 ==
  data: ox_pitch_phi input; ang_term output; ox_lateral_natural_freq input
function ang_term = fcn(ox_pitch_phi, ox_lateral_natural_freq)

ang_term = -ox_lateral_natural_freq^2 * ox_pitch_phi;

end

== matlab function hopper_6dof_NED_v2_fswBridge/Environment/Slosh/Oxidizer Pitch Force/MATLAB Function2 ==
  data: ox_pitch_phi_dot input; velo_term output; ox_lateral_natural_freq input; ox_lateral_damping input
function velo_term = fcn(ox_pitch_phi_dot, ox_lateral_natural_freq,ox_lateral_damping)

velo_term = -2 * ox_lateral_damping * ox_lateral_natural_freq * ox_pitch_phi_dot;
end

== matlab function hopper_6dof_NED_v2_fswBridge/Environment/Slosh/Oxidizer Pitch Force/MATLAB Function3 ==
  data: ox_pitch_phi_ddot input; ox_pitch_f output; ox_lateral_slosh_mass input; ox_lateral_pendulum_l input
function ox_pitch_f = fcn(ox_pitch_phi_ddot, ox_lateral_slosh_mass, ox_lateral_pendulum_l)

ox_pitch_f = ox_lateral_slosh_mass * ox_lateral_pendulum_l * ox_pitch_phi_ddot;
end
